simulink model "simulink_flightgear_control_trim_wind_5"  (R2023a)
settings: Solver=VariableStepAuto  StartTime=0  StopTime=inf  FixedStep=0.1  RelTol=1e-3
values from neighbouring files (symbols this model uses):
  alpha = -5:0.1:25    [Boeing747model.m]
  alpha1 = 0:0.1:14    [Boeing747model.m]
  alpha2 = -5:0.1:25    [Boeing747model.m]
  alpha3 = -5:0.1:17    [Boeing747model.m]
  beta = -15:0.1:15    [Boeing747model.m]
  CL = 0:0.01:1.4    [Boeing747model.m]
  da = 0:1:20    [Boeing747model.m]
  dr = [0 5 10 15 20 25]    [Boeing747model.m]
  EPR_ = 0:0.1:1.8    [Boeing747model.m]    (also in engine.m)
  flap = [0 10 20 25 30]    [Boeing747model.m]
  high1 = 0:10000:40000    [Boeing747model.m]
  high2 = 0:20000:40000    [Boeing747model.m]
  high3 = [0 15000 25000 35000 40000]    [Boeing747model.m]    (also in engine.m)
  high4 = [0 10000 20000 40000]    [Boeing747model.m]
  interp_result = table2array(resultTable(:,2:end))    [Boeing747model.m]
  interp_result_mach = 0:0.1:0.9    [Boeing747model.m]
  interp_result_N1 = 80:5:110    [Boeing747model.m]
  m2ft = 3.280839895013    (= 3.28083989501)    [Boeing747model.m]    (also in engine.m)
  mach = 0:0.02:0.9    [Boeing747model.m]    (also in engine.m)
  mach1 = [0 0.3 0.5 0.7 0.8 0.84 0.86 0.88 0.9]    [Boeing747model.m]
  mach2 = [0 0.3 0.5 0.7 0.8 0.9]    [Boeing747model.m]
  mach3 = [0 0.1 0.3 0.5 0.6 0.7 0.8 0.9]    [Boeing747model.m]    (also in engine.m = [0 0.1 0.3 0.5  0.7 0.8 0.9])
  mach5 = [0 0.6 0.8 0.85 0.9]    [Boeing747model.m]
  mach6 = [0 0.6 0.8 0.9]    [Boeing747model.m]
  mach7 = [0 0.3 0.5 0.74 0.8 0.84 0.86 0.88 0.9]    [Boeing747model.m]
  mach8 = [0 0.3 0.5 0.74 0.8 0.84 0.86 0.88 0.9]    [Boeing747model.m]
  model = 'simulink_flightgear_control_trim_wind_5'    [traimcode.m]
  ms2kts = 1.943844492609    (= 1.94384449261)    [Boeing747model.m]    (also in engine.m)
  powerangle_ = 0:1:130    [Boeing747model.m]    (also in engine.m)
  T = [-45 0 60 120]    [Boeing747model.m]    (also in engine.m)
  V_E = 0:20:250    [Boeing747model.m]
undefined symbols (not defined in the file or in its folder): Earth, F, ft, Light, m, MIL, Model, Newton, P3DAERO, Raphson, Receive, s, Send, Unit, WGS84, Wind
libraries: simulink_extras x115, aerolibconvert2 x16, simulink x4, aerolibfltsims x3, shared6dof x1, aerolibasang x1, aerolibtransform2 x1, aerolibatmos2 x1, aerolibobsolete x1, aerolibwind2 x1
(part 3 of 5)

== system simulink_flightgear_control_trim_wind_5/Plane/参数计算/航迹角/Subsystem3 ==
  Vg : Inport
  Demux2 : Demux  Outputs=3
  Product : Product  RndMeth=Zero
  Product1 : Product  RndMeth=Zero
  Sum : Sum  Inputs=++|
  Terminator1 : Terminator
  Vx²+Vy² : Outport  VectorParamsAs1DForOutWhenUnconnected=off
  wires:
  Product1/1 -> Sum/2
  Demux2/1 -> Product/1, Product/2
  Vg/1 -> Demux2/1
  Demux2/2 -> Product1/1, Product1/2
  Product/1 -> Sum/1
  Sum/1 -> Vx²+Vy²/1
  Demux2/3 -> Terminator1/1

== system simulink_flightgear_control_trim_wind_5/Plane/大气环境/风场_地面坐标系/Subsystem ==
  Vgx : Inport
  WindSpeed : Inport  Port=2
  Abs : Abs  SaturateOnIntegerOverflow=off
  Constant2 : Constant  Value=Wind.Total.Length
  Divide : Product  Inputs=*/
  Rate Limiter Dynamic : simulink/Discontinuities/Rate Limiter Dynamic
  Saturation : Saturate  UpperLimit=inf  LowerLimit=Wind.Total.GrowRate_Min
  Saturation1 : Saturate  UpperLimit=-Wind.Total.GrowRate_Min  LowerLimit=-inf
  Unary Minus : UnaryMinus
  V_Wind : Outport  VectorParamsAs1DForOutWhenUnconnected=off
  wires:
  Saturation1/1 -> Rate Limiter Dynamic/3
  Saturation/1 -> Rate Limiter Dynamic/1
  Abs/1 -> Divide/1
  Unary Minus/1 -> Saturation1/1
  Vgx/1 -> Abs/1
  Divide/1 -> Saturation/1, Unary Minus/1
  Constant2/1 -> Divide/2
  WindSpeed/1 -> Rate Limiter Dynamic/2
  Rate Limiter Dynamic/1 -> V_Wind/1

== system simulink_flightgear_control_trim_wind_5/Plane/大气环境/风场_地面坐标系/常值风 ==
  h(m) : Inport
  Constant : Constant  Value=0
  Fcn : Fcn  Expr=Wind.Constant.Vxy_Ground + (Wind.Constant.Vxy_RefAlt / Wind.Constant.RefAlt^2)
  Gain : Gain  Gain=cos(deg2rad(Wind.Constant.Direction))
  Gain1 : Gain  Gain=sin(deg2rad(Wind.Constant.Direction))
  Mux : Mux  Inputs=3
  V_Wind_Constant : Outport  VectorParamsAs1DForOutWhenUnconnected=off
  wires:
  Mux/1 -> V_Wind_Constant/1
  Gain1/1 -> Mux/2
  Constant/1 -> Mux/3
  Fcn/1 -> Gain/1, Gain1/1
  Gain/1 -> Mux/1
  h(m)/1 -> Fcn/1

== system simulink_flightgear_control_trim_wind_5/Plane/大气环境/风场_地面坐标系/自定义 ==
  Angle Conversion2 : aerolibconvert2/Angle Conversion  IU=deg  OU=rad
  Mux : Mux  Inputs=3
  Product : Product
  Product1 : Product
  Trigonometric Function : Trigonometry  Operator=cos
  Trigonometric Function1 : Trigonometry
  Wind_Custom_Direction : Constant  Value=Wind.Custom.Direction
  Wind_Custom_Vxy : Constant  Value=Wind.Custom.Vxy
  Wind_Custom_Vz : Constant  Value=Wind.Custom.Vz
  V_Wind_Custom : Outport  VectorParamsAs1DForOutWhenUnconnected=off
  wires:
  Angle Conversion2/1 -> Trigonometric Function/1, Trigonometric Function1/1
  Wind_Custom_Vxy/1 -> Product/1, Product1/1
  Trigonometric Function/1 -> Product/2
  Trigonometric Function1/1 -> Product1/2
  Wind_Custom_Direction/1 -> Angle Conversion2/1
  Product/1 -> Mux/1
  Wind_Custom_Vz/1 -> Mux/3
  Product1/1 -> Mux/2
  Mux/1 -> V_Wind_Custom/1

== system simulink_flightgear_control_trim_wind_5/Plane/大气环境/风场_地面坐标系/阵风 ==
  Angle Conversion1 : aerolibconvert2/Angle Conversion  IU=deg  OU=rad
  Constant1 : Constant  Value=Wind.Gust.Vxy_max
  Constant2 : Constant  Value=Wind.Gust.Vz_max
  Constant3 : Constant  Value=Wind.Gust.Act_Random_V
  Constant4 : Constant  Value=Wind.Gust.Direction
  Constant6 : Constant  Value=Wind.Gust.Act_Random_Direction
  Constant7 : Constant  Value=Wind.Gust.Act_Random_V
  Mux : Mux  Inputs=3
  Product : Product
  Product3 : Product
  Product4 : Product
  Pulse Generator : DiscretePulseGenerator  PulseType=Time based  Period=Wind.Gust.SampleTime + Wind.Gust.ContinueTime  PulseWidth=Wind.Gust.ContinueTime / (Wind.Gust.SampleTime + Wind.Gust.ContinueTime) * 100  PhaseDelay=Wind.Gust.SampleTime
  Switch : Switch  Criteria=u2 ~= 0  SaturateOnIntegerOverflow=off  InputSameDT=off
  Switch1 : Switch  Criteria=u2 ~= 0  SaturateOnIntegerOverflow=off  InputSameDT=off
  Switch2 : Switch  Criteria=u2 ~= 0  SaturateOnIntegerOverflow=off  InputSameDT=off
  Trigonometric Function : Trigonometry  Operator=cos
  Trigonometric Function1 : Trigonometry
  Uniform Random Number : UniformRandomNumber  Minimum=Wind.Gust.Vxy_min  Maximum=Wind.Gust.Vxy_max + eps  Seed=fix(rand(1,1)*25000)  SampleTime=Wind.Gust.SampleTime + Wind.Gust.ContinueTime
  Uniform Random Number1 : UniformRandomNumber  Minimum=0  Maximum=360  Seed=fix(rand(1,1)*25000)  SampleTime=Wind.Gust.SampleTime + Wind.Gust.ContinueTime
  Uniform Random Number2 : UniformRandomNumber  Minimum=Wind.Gust.Vz_min  Maximum=Wind.Gust.Vz_max + eps  Seed=fix(rand(1,1)*25000)  SampleTime=Wind.Gust.SampleTime + Wind.Gust.ContinueTime
  V_Wind_Gust : Outport  VectorParamsAs1DForOutWhenUnconnected=off
  wires:
  Uniform Random Number2/1 -> Switch2/1
  Constant7/1 -> Switch2/2
  Angle Conversion1/1 -> Trigonometric Function/1, Trigonometric Function1/1
  Constant4/1 -> Switch1/3
  Uniform Random Number1/1 -> Switch1/1
  Constant6/1 -> Switch1/2
  Trigonometric Function1/1 -> Product4/2
  Trigonometric Function/1 -> Product/2
  Switch/1 -> Product/1, Product4/1
  Switch1/1 -> Angle Conversion1/1
  Mux/1 -> Product3/1
  Constant2/1 -> Switch2/3
  Constant3/1 -> Switch/2
  Switch2/1 -> Mux/3
  Uniform Random Number/1 -> Switch/1
  Constant1/1 -> Switch/3
  Pulse Generator/1 -> Product3/2
  Product4/1 -> Mux/2
  Product/1 -> Mux/1
  Product3/1 -> V_Wind_Gust/1

== system simulink_flightgear_control_trim_wind_5/Plane/气动系数/Subsystem58/Subsystem ==
  note: 高速模式
  In1 : Inport
  Radians in : Inport  Port=2
  In3 : Inport  Port=3
  2-D Lookup Table3 : Lookup_n-D  BreakpointsForDimension1=mach7  BreakpointsForDimension2=alpha2  Table=P3DAERO.CL_mach  InternalRulePriority=Speed  RndMeth=Simplest
      settings: InputPortMap=u0,u1
  Radians to Degrees : simulink_extras/Transformations/Radians to Degrees
  Scope2 : Scope
  Out1 : Outport
  wires:
  Radians in/1 -> Radians to Degrees/1
  Radians to Degrees/1 -> 2-D Lookup Table3/2
  In3/1 -> 2-D Lookup Table3/1
  2-D Lookup Table3/1 -> Scope2/1, Out1/1

== system simulink_flightgear_control_trim_wind_5/Plane/气动系数/Subsystem58/Subsystem1 ==
  note: 高速模式
  note: 低速模式
  In1 : Inport
  In2 : Inport  Port=2
  In3 : Inport  Port=3
  In4 : Inport  Port=4
  2-D Lookup Table19 : Lookup_n-D  BreakpointsForDimension1=flap  BreakpointsForDimension2=V_E  Table=P3DAERO.Delta_CL_lowspeed  InternalRulePriority=Speed  RndMeth=Simplest
      settings: InputPortMap=u0,u1
  2-D Lookup Table20 : Lookup_n-D  BreakpointsForDimension1=high1  BreakpointsForDimension2=mach  Table=P3DAERO.Delta_CL_highspeed  InternalRulePriority=Speed  RndMeth=Simplest
      settings: InputPortMap=u0,u1
  Gain11 : Gain  Gain=-1
  Scope6 : Scope
  Velocity Conversion : aerolibconvert2/Velocity Conversion  IU=m/s  OU=ft/s
  Out1 : Outport
  wires:
  2-D Lookup Table20/1 -> Gain11/1
  Gain11/1 -> Out1/1, Scope6/1
  In4/1 -> 2-D Lookup Table20/2
  In2/1 -> 2-D Lookup Table19/2
  In3/1 -> Velocity Conversion/1
  In1/1 -> 2-D Lookup Table19/1
  Velocity Conversion/1 -> 2-D Lookup Table20/1

== system simulink_flightgear_control_trim_wind_5/Plane/气动系数/Subsystem58/Subsystem10 ==
  note: dot_CL_dot_delta_ei
  In1 : Inport
  In2 : Inport  Port=2
  In3 : Inport  Port=3
  Radians in : Inport  Port=4
  2-D Lookup Table10 : Lookup_n-D  BreakpointsForDimension1=high1  BreakpointsForDimension2=mach  Table=P3DAERO.dot_CL_dot_delta_ei  InternalRulePriority=Speed  RndMeth=Simplest
      settings: InputPortMap=u0,u1
  Gain : Gain
  Product6 : Product  Inputs=3
  Radians to Degrees4 : simulink_extras/Transformations/Radians to Degrees
  Scope1 : Scope
  Scope18 : Scope
  Velocity Conversion : aerolibconvert2/Velocity Conversion  IU=m/s  OU=ft/s
  Out1 : Outport
  wires:
  Product6/1 -> Gain/1, Scope18/1
  Radians in/1 -> Radians to Degrees4/1
  In1/1 -> Product6/1
  Radians to Degrees4/1 -> Product6/3, Scope1/1
  2-D Lookup Table10/1 -> Product6/2
  In3/1 -> 2-D Lookup Table10/2
  In2/1 -> Velocity Conversion/1
  Gain/1 -> Out1/1
  Velocity Conversion/1 -> 2-D Lookup Table10/1

== system simulink_flightgear_control_trim_wind_5/Plane/气动系数/Subsystem58/Subsystem12 ==
  In1 : Inport
  Radians in : Inport  Port=2
  2-D Lookup Table : Lookup_n-D  BreakpointsForDimension1=flap  BreakpointsForDimension2=alpha  Table=P3DAERO.CD_basic  InternalRulePriority=Speed  RndMeth=Simplest
      settings: InputPortMap=u0,u1
  Radians to Degrees : simulink_extras/Transformations/Radians to Degrees
  Scope14 : Scope
  Out1 : Outport
  wires:
  In1/1 -> 2-D Lookup Table/1
  Radians to Degrees/1 -> 2-D Lookup Table/2
  2-D Lookup Table/1 -> Out1/1, Scope14/1
  Radians in/1 -> Radians to Degrees/1

== system simulink_flightgear_control_trim_wind_5/Plane/气动系数/Subsystem58/Subsystem13 ==
  In1 : Inport
  Radians in : Inport  Port=2
  Radians in1 : Inport  Port=3
  2-D Lookup Table1 : Lookup_n-D  BreakpointsForDimension1=flap  BreakpointsForDimension2=alpha  Table=P3DAERO.dot_CD_dot_delta  InternalRulePriority=Speed  RndMeth=Simplest
      settings: InputPortMap=u0,u1
  Product : Product
  Radians to Degrees2 : simulink_extras/Transformations/Radians to Degrees
  Radians to Degrees7 : simulink_extras/Transformations/Radians to Degrees
  Scope5 : Scope
  Out1 : Outport
  wires:
  Radians in1/1 -> Radians to Degrees2/1
  Product/1 -> Out1/1, Scope5/1
  Radians to Degrees2/1 -> Product/2
  2-D Lookup Table1/1 -> Product/1
  Radians to Degrees7/1 -> 2-D Lookup Table1/2
  In1/1 -> 2-D Lookup Table1/1
  Radians in/1 -> Radians to Degrees7/1

== system simulink_flightgear_control_trim_wind_5/Plane/气动系数/Subsystem58/Subsystem14 ==
  In1 : Inport
  In2 : Inport  Port=2
  In3 : Inport  Port=3
  In4 : Inport  Port=4
  In5 : Inport  Port=5
  2-D Lookup Table2 : Lookup_n-D  BreakpointsForDimension1=mach1  BreakpointsForDimension2=CL  Table=P3DAERO.CD_mach  InternalRulePriority=Speed  RndMeth=Simplest
      settings: InputPortMap=u0,u1
  Gain : Gain
  Scope : Scope
  Scope2 : Scope
  Sum2 : Sum
  Out1 : Outport
  wires:
  In4/1 -> 2-D Lookup Table2/1
  2-D Lookup Table2/1 -> Gain/1
  In5/1 -> 2-D Lookup Table2/2
  Gain/1 -> Scope/1, Out1/1
  Sum2/1 -> Scope2/1
  In1/1 -> Sum2/1
  In2/1 -> Sum2/2

== system simulink_flightgear_control_trim_wind_5/Plane/气动系数/Subsystem58/Subsystem15 ==
  Radians in : Inport
  In2 : Inport  Port=2
  2-D Lookup Table6 : Lookup_n-D  BreakpointsForDimension1=dr  BreakpointsForDimension2=beta  Table=P3DAERO.delta_CD_25R  InternalRulePriority=Speed  RndMeth=Simplest
      settings: InputPortMap=u0,u1
  2-D Lookup Table9 : Lookup_n-D  BreakpointsForDimension1=dr  BreakpointsForDimension2=beta  Table=P3DAERO.delta_CD_fu25R  InternalRulePriority=Speed  RndMeth=Simplest
      settings: InputPortMap=u0,u1
  Abs1 : Abs  SaturateOnIntegerOverflow=off
  Gain4 : Gain  Gain=0.6
  Gain8 : Gain  Gain=0.6
  Radians to Degrees{6,8..9,11} (4 alike) : simulink_extras/Transformations/Radians to Degrees
  Saturation1 : Saturate  UpperLimit=15  LowerLimit=-15
  Saturation9 : Saturate  UpperLimit=15  LowerLimit=-15
  Scope17 : Scope
  Switch2 : Switch  SaturateOnIntegerOverflow=off  InputSameDT=off
  Out1 : Outport
  wires:
  Radians to Degrees9/1 -> Abs1/1
  Radians in/1 -> Radians to Degrees8/1, Radians to Degrees6/1
  In2/1 -> Radians to Degrees9/1, Radians to Degrees11/1, Switch2/2
  2-D Lookup Table6/1 -> Gain4/1, Scope17/1
  Gain4/1 -> Switch2/1
  Gain8/1 -> Switch2/3
  Saturation9/1 -> 2-D Lookup Table6/2
  Radians to Degrees6/1 -> Saturation9/1
  2-D Lookup Table9/1 -> Gain8/1
  Radians to Degrees8/1 -> Saturation1/1
  Radians to Degrees11/1 -> 2-D Lookup Table6/1
  Switch2/1 -> Out1/1
  Abs1/1 -> 2-D Lookup Table9/1
  Saturation1/1 -> 2-D Lookup Table9/2

== system simulink_flightgear_control_trim_wind_5/Plane/气动系数/Subsystem58/Subsystem16 ==
  Radians in : Inport
  In2 : Inport  Port=2
  2-D Lookup Table7 : Lookup_n-D  BreakpointsForDimension1=dr  BreakpointsForDimension2=beta  Table=P3DAERO.delta_CD_25R  InternalRulePriority=Speed  RndMeth=Simplest
      settings: InputPortMap=u0,u1
  2-D Lookup Table8 : Lookup_n-D  BreakpointsForDimension1=dr  BreakpointsForDimension2=beta  Table=P3DAERO.delta_CD_fu25R  InternalRulePriority=Speed  RndMeth=Simplest
      settings: InputPortMap=u0,u1
  Abs2 : Abs  SaturateOnIntegerOverflow=off
  Gain10 : Gain  Gain=0.4
  Gain12 : Gain  Gain=0.4
  Radians to Degrees{5,10,12..13} (4 alike) : simulink_extras/Transformations/Radians to Degrees
  Saturation1 : Saturate  UpperLimit=15  LowerLimit=-15
  Saturation10 : Saturate  UpperLimit=15  LowerLimit=-15
  Scope11 : Scope
  Switch3 : Switch  SaturateOnIntegerOverflow=off  InputSameDT=off
  Out1 : Outport
  wires:
  Gain10/1 -> Scope11/1, Switch3/1
  Radians in/1 -> Radians to Degrees12/1, Radians to Degrees5/1
  Radians to Degrees12/1 -> Saturation1/1
  In2/1 -> Radians to Degrees13/1, Radians to Degrees10/1, Switch3/2
  Radians to Degrees13/1 -> Abs2/1
  Gain12/1 -> Switch3/3
  Saturation10/1 -> 2-D Lookup Table7/2
  2-D Lookup Table7/1 -> Gain10/1
  Radians to Degrees5/1 -> Saturation10/1
  Radians to Degrees10/1 -> 2-D Lookup Table7/1
  2-D Lookup Table8/1 -> Gain12/1
  Switch3/1 -> Out1/1
  Abs2/1 -> 2-D Lookup Table8/1
  Saturation1/1 -> 2-D Lookup Table8/2

== system simulink_flightgear_control_trim_wind_5/Plane/气动系数/Subsystem58/Subsystem17 ==
  note: 米变英尺
  In1 : Inport
  In2 : Inport  Port=2
  Radians in : Inport  Port=3
  1-D Lookup Table97 : Lookup_n-D  NumberOfTableDimensions=1  BreakpointsForDimension1=P3DAERO.k_ge_A(1,:)  Table=P3DAERO.k_ge_A(2,:)  InternalRulePriority=Speed  RndMeth=Simplest
  2-D Lookup Table4 : Lookup_n-D  BreakpointsForDimension1=flap  BreakpointsForDimension2=alpha1  Table=P3DAERO.delta_CD_ge  InternalRulePriority=Speed  RndMeth=Simplest
      settings: InputPortMap=u0,u1
  Constant24 : Constant  Value=0
  Gain : Gain
  Product1 : Product
  Radians to Degrees3 : simulink_extras/Transformations/Radians to Degrees
  Saturation1 : Saturate  UpperLimit=14  LowerLimit=0
  Scope15 : Scope
  Scope49 : Scope
  Switch12 : Switch  Criteria=u2 > Threshold  Threshold=24  SaturateOnIntegerOverflow=off  InputSameDT=off
  Velocity Conversion : aerolibconvert2/Velocity Conversion  IU=m/s  OU=ft/s
  Out1 : Outport
  wires:
  Saturation1/1 -> 2-D Lookup Table4/2
  Switch12/1 -> Gain/1, Scope49/1
  Radians to Degrees3/1 -> Saturation1/1
  1-D Lookup Table97/1 -> Product1/1
  Velocity Conversion/1 -> 1-D Lookup Table97/1
  Product1/1 -> Switch12/3
  Radians in/1 -> Radians to Degrees3/1
  2-D Lookup Table4/1 -> Scope15/1, Product1/2
  In2/1 -> 2-D Lookup Table4/1
  Constant24/1 -> Switch12/1
  Gain/1 -> Out1/1
  In1/1 -> Switch12/2, Velocity Conversion/1

== system simulink_flightgear_control_trim_wind_5/Plane/气动系数/Subsystem58/Subsystem18 ==
  In1 : Inport
  Radians in : Inport  Port=2
  2-D Lookup Table5 : Lookup_n-D  BreakpointsForDimension1=flap  BreakpointsForDimension2=beta  Table=P3DAERO.delta_CD_sideslip  InternalRulePriority=Speed  RndMeth=Simplest
      settings: InputPortMap=u0,u1
  Gain1 : Gain  Gain=-1
  Radians to Degrees4 : simulink_extras/Transformations/Radians to Degrees
  Saturation8 : Saturate  UpperLimit=15  LowerLimit=-15
  Scope16 : Scope
  Out1 : Outport
  wires:
  Gain1/1 -> Out1/1, Scope16/1
  Radians to Degrees4/1 -> Saturation8/1
  Saturation8/1 -> 2-D Lookup Table5/2
  In1/1 -> 2-D Lookup Table5/1
  2-D Lookup Table5/1 -> Gain1/1
  Radians in/1 -> Radians to Degrees4/1

== system simulink_flightgear_control_trim_wind_5/Plane/气动系数/Subsystem58/Subsystem19 ==
  In1 : Inport
  In2 : Inport  Port=2
  Radians in : Inport  Port=3
  In4 : Inport  Port=4
  1-D Lookup Table91 : Lookup_n-D  NumberOfTableDimensions=1  BreakpointsForDimension1=P3DAERO.CD_mach_gear(1,:)  Table=P3DAERO.CD_mach_gear(2,:)  InternalRulePriority=Speed  RndMeth=Simplest
  2-D Lookup Table3 : Lookup_n-D  BreakpointsForDimension1=flap  BreakpointsForDimension2=alpha  Table=P3DAERO.delta_CD_gear  InternalRulePriority=Speed  RndMeth=Simplest
      settings: InputPortMap=u0,u1
  Product15 : Product  Inputs=3
  Radians to Degrees2 : simulink_extras/Transformations/Radians to Degrees
  Scope17 : Scope
  Scope47 : Scope
  Out1 : Outport
  wires:
  Product15/1 -> Out1/1, Scope47/1
  In2/1 -> 2-D Lookup Table3/1
  2-D Lookup Table3/1 -> Product15/2
  Radians to Degrees2/1 -> 2-D Lookup Table3/2
  In1/1 -> Product15/1
  1-D Lookup Table91/1 -> Scope17/1, Product15/3
  In4/1 -> 1-D Lookup Table91/1
  Radians in/1 -> Radians to Degrees2/1

== system simulink_flightgear_control_trim_wind_5/Plane/气动系数/Subsystem58/Subsystem2 ==
  note: dot_CL_dot_delta_eo
  In1 : Inport
  In2 : Inport  Port=2
  In3 : Inport  Port=3
  Radians in : Inport  Port=4
  2-D Lookup Table11 : Lookup_n-D  BreakpointsForDimension1=high1  BreakpointsForDimension2=mach  Table=P3DAERO.dot_CL_dot_delta_eo  InternalRulePriority=Speed  RndMeth=Simplest
      settings: InputPortMap=u0,u1
  Gain : Gain
  Product7 : Product  Inputs=3
  Radians to Degrees5 : simulink_extras/Transformations/Radians to Degrees
  Scope1 : Scope
  Scope19 : Scope
  Velocity Conversion : aerolibconvert2/Velocity Conversion  IU=m/s  OU=ft/s
  Out1 : Outport
  wires:
  Radians to Degrees5/1 -> Scope1/1, Product7/3
  In3/1 -> 2-D Lookup Table11/2
  Product7/1 -> Gain/1, Scope19/1
  In1/1 -> Product7/1
  2-D Lookup Table11/1 -> Product7/2
  Radians in/1 -> Radians to Degrees5/1
  In2/1 -> Velocity Conversion/1
  Gain/1 -> Out1/1
  Velocity Conversion/1 -> 2-D Lookup Table11/1

== system simulink_flightgear_control_trim_wind_5/Plane/气动系数/Subsystem58/Subsystem20 ==
  In1 : Inport
  Radians in : Inport  Port=2
  In3 : Inport  Port=3
  2-D Lookup Table : Lookup_n-D  BreakpointsForDimension1=flap  BreakpointsForDimension2=alpha  Table=P3DAERO.Cm_25_basic  InternalRulePriority=Speed  RndMeth=Simplest
      settings: InputPortMap=u0,u1
  2-D Lookup Table1 : Lookup_n-D  BreakpointsForDimension1=mach8  BreakpointsForDimension2=alpha3  Table=P3DAERO.Cm_mach  InternalRulePriority=Speed  RndMeth=Simplest
      settings: InputPortMap=u0,u1
  Radians to Degrees6 : simulink_extras/Transformations/Radians to Degrees
  Saturation : Saturate  UpperLimit=17  LowerLimit=-5
  Scope : Scope
  Scope2 : Scope
  Scope3 : Scope
  Out1 : Outport
  wires:
  Saturation/1 -> Scope3/1, 2-D Lookup Table1/2
  In3/1 -> 2-D Lookup Table1/1
  In1/1 -> 2-D Lookup Table/1
  2-D Lookup Table1/1 -> Scope2/1, Out1/1
  Radians in/1 -> Radians to Degrees6/1
  Radians to Degrees6/1 -> Saturation/1, 2-D Lookup Table/2
  2-D Lookup Table/1 -> Scope/1

== system simulink_flightgear_control_trim_wind_5/Plane/气动系数/Subsystem58/Subsystem21 ==
  note: 低速模式
  note: 高速模式
  In1 : Inport
  In2 : Inport  Port=2
  In3 : Inport  Port=3
  In4 : Inport  Port=4
  2-D Lookup Table1 : Lookup_n-D  BreakpointsForDimension1=high1  BreakpointsForDimension2=mach  Table=P3DAERO.delta_Cm_25_highspeed  InternalRulePriority=Speed  RndMeth=Simplest
      settings: InputPortMap=u0,u1
  2-D Lookup Table2 : Lookup_n-D  BreakpointsForDimension1=flap  BreakpointsForDimension2=V_E  Table=P3DAERO.delta_Cm_25_lowspeed  InternalRulePriority=Speed  RndMeth=Simplest
      settings: InputPortMap=u0,u1
  Gain7 : Gain  Gain=m2ft
  Scope2 : Scope
  Out1 : Outport
  wires:
  In2/1 -> 2-D Lookup Table2/2
  Gain7/1 -> 2-D Lookup Table1/1
  In3/1 -> Gain7/1
  In1/1 -> 2-D Lookup Table2/1
  2-D Lookup Table1/1 -> Out1/1, Scope2/1
  In4/1 -> 2-D Lookup Table1/2

== system simulink_flightgear_control_trim_wind_5/Plane/气动系数/Subsystem58/Subsystem22 ==
  note: 地效修正
  note: 米变英尺
  In1 : Inport
  In2 : Inport  Port=2
  Radians in : Inport  Port=3
  1-D Lookup Table97 : Lookup_n-D  NumberOfTableDimensions=1  BreakpointsForDimension1=P3DAERO.k_ge(1,:)  Table=P3DAERO.k_ge(2,:)  InternalRulePriority=Speed  RndMeth=Simplest
  2-D Lookup Table13 : Lookup_n-D  BreakpointsForDimension1=flap  BreakpointsForDimension2=alpha1  Table=P3DAERO.Fm  InternalRulePriority=Speed  RndMeth=Simplest
      settings: InputPortMap=u0,u1
  Constant21 : Constant
  Gain14 : Gain  Gain=m2ft
  Product16 : Product
  Radians to Degrees2 : simulink_extras/Transformations/Radians to Degrees
  Saturation : Saturate  UpperLimit=14  LowerLimit=0
  Scope31 : Scope
  Scope48 : Scope
  Sum11 : Sum
  Switch5 : Switch  Criteria=u2 > Threshold  Threshold=24  SaturateOnIntegerOverflow=off  InputSameDT=off
  Out1 : Outport
  wires:
  Saturation/1 -> 2-D Lookup Table13/2
  Gain14/1 -> 1-D Lookup Table97/1
  Product16/1 -> Sum11/2
  Switch5/1 -> Out1/1, Scope31/1
  Radians to Degrees2/1 -> Saturation/1
  2-D Lookup Table13/1 -> Product16/2
  Sum11/1 -> Switch5/3
  Radians in/1 -> Radians to Degrees2/1
  Constant21/1 -> Sum11/1, Switch5/1
  1-D Lookup Table97/1 -> Scope48/1, Product16/1
  In2/1 -> 2-D Lookup Table13/1
  In1/1 -> Switch5/2, Gain14/1

== system simulink_flightgear_control_trim_wind_5/Plane/气动系数/Subsystem58/Subsystem23 ==
  In1 : Inport
  Radians in : Inport  Port=2
  In3 : Inport  Port=3
  Radians in1 : Inport  Port=4
  In5 : Inport  Port=5
  1-D Lookup Table1 : Lookup_n-D  NumberOfTableDimensions=1  BreakpointsForDimension1=P3DAERO.delta_CM_25_ai_flapup(1,:)  Table=P3DAERO.delta_CM_25_ai_flapup(2,:)  InternalRulePriority=Speed  RndMeth=Simplest
  1-D Lookup Table2 : Lookup_n-D  NumberOfTableDimensions=1  BreakpointsForDimension1=P3DAERO.delta_CM_25_ai_flapdown(1,:)  Table=P3DAERO.delta_CM_25_ai_flapdown(2,:)  InternalRulePriority=Speed  RndMeth=Simplest
  1-D Lookup Table35 : Lookup_n-D  NumberOfTableDimensions=1  BreakpointsForDimension1=P3DAERO.delta_CM_25_ai_mach(1,:)  Table=P3DAERO.delta_CM_25_ai_mach(2,:)  InternalRulePriority=Speed  RndMeth=Simplest
  2-D Lookup Table14 : Lookup_n-D  BreakpointsForDimension1=flap  BreakpointsForDimension2=da  Table=P3DAERO.k_delta_ai  InternalRulePriority=Speed  RndMeth=Simplest
      settings: InputPortMap=u0,u1
  Product4 : Product  Inputs=4
  Radians to Degrees4 : simulink_extras/Transformations/Radians to Degrees
  Radians to Degrees8 : simulink_extras/Transformations/Radians to Degrees
  Saturation2 : Saturate  UpperLimit=20  LowerLimit=0
  Scope15 : Scope
  Switch15 : Switch  Criteria=u2 ~= 0  Threshold=0.35  SaturateOnIntegerOverflow=off  InputSameDT=off
  Out1 : Outport
  wires:
  Radians to Degrees4/1 -> Saturation2/1
  1-D Lookup Table1/1 -> Switch15/3
  1-D Lookup Table2/1 -> Switch15/1
  2-D Lookup Table14/1 -> Product4/3
  Switch15/1 -> Product4/2
  In1/1 -> 1-D Lookup Table35/1
  Saturation2/1 -> 2-D Lookup Table14/2
  In3/1 -> Switch15/2, 2-D Lookup Table14/1
  Product4/1 -> Out1/1, Scope15/1
  Radians to Degrees8/1 -> 1-D Lookup Table2/1, 1-D Lookup Table1/1
  In5/1 -> Product4/4
  1-D Lookup Table35/1 -> Product4/1
  Radians in/1 -> Radians to Degrees8/1
  Radians in1/1 -> Radians to Degrees4/1

== system simulink_flightgear_control_trim_wind_5/Plane/气动系数/Subsystem58/Subsystem24 ==
  In1 : Inport
  Radians in : Inport  Port=2
  In3 : Inport  Port=3
  Radians in1 : Inport  Port=4
  In5 : Inport  Port=5
  1-D Lookup Table3 : Lookup_n-D  NumberOfTableDimensions=1  BreakpointsForDimension1=P3DAERO.delta_CM_25_ai_flapup(1,:)  Table=P3DAERO.delta_CM_25_ai_flapup(2,:)  InternalRulePriority=Speed  RndMeth=Simplest
  1-D Lookup Table4 : Lookup_n-D  NumberOfTableDimensions=1  BreakpointsForDimension1=P3DAERO.delta_CM_25_ai_flapdown(1,:)  Table=P3DAERO.delta_CM_25_ai_flapdown(2,:)  InternalRulePriority=Speed  RndMeth=Simplest
  1-D Lookup Table5 : Lookup_n-D  NumberOfTableDimensions=1  BreakpointsForDimension1=P3DAERO.delta_CM_25_ai_mach(1,:)  Table=P3DAERO.delta_CM_25_ai_mach(2,:)  InternalRulePriority=Speed  RndMeth=Simplest
  2-D Lookup Table15 : Lookup_n-D  BreakpointsForDimension1=flap  BreakpointsForDimension2=da  Table=P3DAERO.k_delta_ai  InternalRulePriority=Speed  RndMeth=Simplest
      settings: InputPortMap=u0,u1
  Product18 : Product  Inputs=4
  Radians to Degrees16 : simulink_extras/Transformations/Radians to Degrees
  Radians to Degrees9 : simulink_extras/Transformations/Radians to Degrees
  Saturation4 : Saturate  UpperLimit=20  LowerLimit=0
  Scope6 : Scope
  Switch16 : Switch  Criteria=u2 ~= 0  Threshold=0.35  SaturateOnIntegerOverflow=off  InputSameDT=off
  Out1 : Outport
  wires:
  Switch16/1 -> Product18/2
  Radians to Degrees9/1 -> Saturation4/1
  Saturation4/1 -> 2-D Lookup Table15/2
  1-D Lookup Table5/1 -> Product18/1
  In5/1 -> Product18/4
  1-D Lookup Table4/1 -> Switch16/1
  In3/1 -> 2-D Lookup Table15/1, Switch16/2
  Radians to Degrees16/1 -> 1-D Lookup Table4/1, 1-D Lookup Table3/1
  Product18/1 -> Out1/1, Scope6/1
  Radians in/1 -> Radians to Degrees16/1
  1-D Lookup Table3/1 -> Switch16/3
  2-D Lookup Table15/1 -> Product18/3
  In1/1 -> 1-D Lookup Table5/1
  Radians in1/1 -> Radians to Degrees9/1

== system simulink_flightgear_control_trim_wind_5/Plane/气动系数/Subsystem58/Subsystem25 ==
  note: 米变英尺
  In1 : Inport
  In2 : Inport  Port=2
  Radians in : Inport  Port=3
  1-D Lookup Table59 : Lookup_n-D  NumberOfTableDimensions=1  BreakpointsForDimension1=P3DAERO.k_ge(1,:)  Table=P3DAERO.k_ge(2,:)  InternalRulePriority=Speed  RndMeth=Simplest
  2-D Lookup Table21 : Lookup_n-D  BreakpointsForDimension1=flap  BreakpointsForDimension2=alpha1  Table=P3DAERO.delta_CM_25_ge  InternalRulePriority=Speed  RndMeth=Simplest
      settings: InputPortMap=u0,u1
  Constant24 : Constant  Value=0
  Gain3 : Gain  Gain=m2ft
  Product8 : Product
  Radians to Degrees14 : simulink_extras/Transformations/Radians to Degrees
  Saturation5 : Saturate  UpperLimit=14  LowerLimit=0
  Scope11 : Scope
  Scope49 : Scope
  Switch12 : Switch  Criteria=u2 > Threshold  Threshold=24  SaturateOnIntegerOverflow=off  InputSameDT=off
  Out1 : Outport
  wires:
  2-D Lookup Table21/1 -> Product8/2
  Constant24/1 -> Switch12/1
  Switch12/1 -> Out1/1, Scope49/1
  Radians to Degrees14/1 -> Saturation5/1
  Gain3/1 -> 1-D Lookup Table59/1
  1-D Lookup Table59/1 -> Product8/1, Scope11/1
  Product8/1 -> Switch12/3
  Saturation5/1 -> 2-D Lookup Table21/2
  Radians in/1 -> Radians to Degrees14/1
  In2/1 -> 2-D Lookup Table21/1
  In1/1 -> Switch12/2, Gain3/1

== system simulink_flightgear_control_trim_wind_5/Plane/气动系数/Subsystem58/Subsystem26 ==
  In1 : Inport
  Radians in : Inport  Port=2
  2-D Lookup Table22 : Lookup_n-D  BreakpointsForDimension1=flap  BreakpointsForDimension2=beta  Table=P3DAERO.delta_CM_25_sideslip  InternalRulePriority=Speed  RndMeth=Simplest
      settings: InputPortMap=u0,u1
  Radians to Degrees18 : simulink_extras/Transformations/Radians to Degrees
  Scope13 : Scope
  Out1 : Outport
  wires:
  In1/1 -> 2-D Lookup Table22/1
  2-D Lookup Table22/1 -> Out1/1, Scope13/1
  Radians to Degrees18/1 -> 2-D Lookup Table22/2
  Radians in/1 -> Radians to Degrees18/1

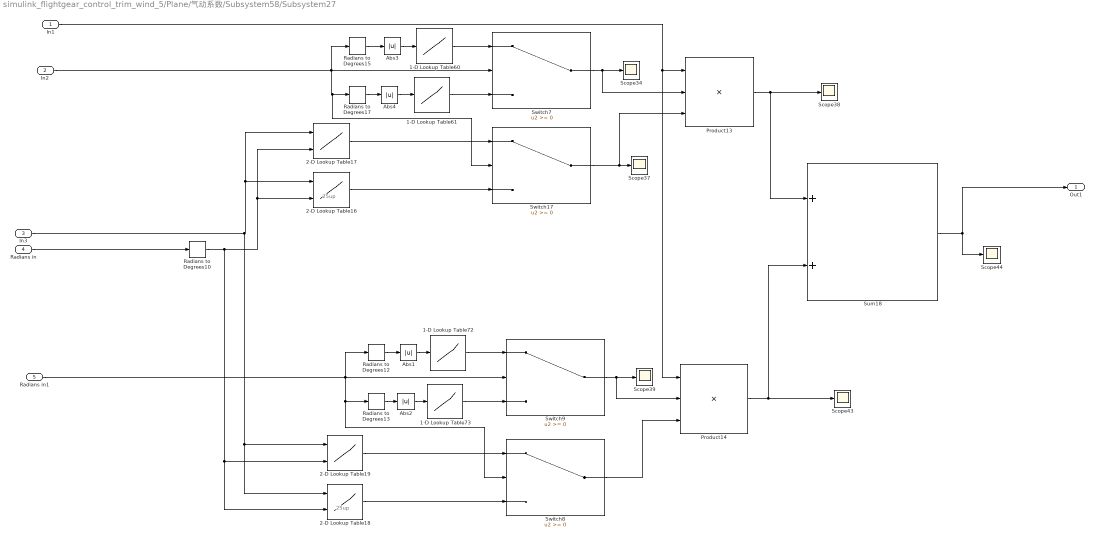
== system simulink_flightgear_control_trim_wind_5/Plane/气动系数/Subsystem58/Subsystem27 ==
  note: 25up
  note: 25up
  In1 : Inport
  In2 : Inport  Port=2
  In3 : Inport  Port=3
  Radians in : Inport  Port=4
  Radians in1 : Inport  Port=5
  1-D Lookup Table60 : Lookup_n-D  NumberOfTableDimensions=1  BreakpointsForDimension1=P3DAERO.k_delata_Ao_down(1,:)  Table=P3DAERO.k_delata_Ao_down(2,:)  InternalRulePriority=Speed  RndMeth=Simplest
  1-D Lookup Table61 : Lookup_n-D  NumberOfTableDimensions=1  BreakpointsForDimension1=P3DAERO.k_delata_Ao_up(1,:)  Table=P3DAERO.k_delata_Ao_up(2,:)  InternalRulePriority=Speed  RndMeth=Simplest
  1-D Lookup Table72 : Lookup_n-D  NumberOfTableDimensions=1  BreakpointsForDimension1=P3DAERO.k_delata_Ao_down(1,:)  Table=P3DAERO.k_delata_Ao_down(2,:)  InternalRulePriority=Speed  RndMeth=Simplest
  1-D Lookup Table73 : Lookup_n-D  NumberOfTableDimensions=1  BreakpointsForDimension1=P3DAERO.k_delata_Ao_up(1,:)  Table=P3DAERO.k_delata_Ao_up(2,:)  InternalRulePriority=Speed  RndMeth=Simplest
  2-D Lookup Table16 : Lookup_n-D  BreakpointsForDimension1=flap  BreakpointsForDimension2=alpha  Table=P3DAERO.delata_CM_25_Ao_25up  InternalRulePriority=Speed  RndMeth=Simplest
      settings: InputPortMap=u0,u1
  2-D Lookup Table17 : Lookup_n-D  BreakpointsForDimension1=flap  BreakpointsForDimension2=alpha  Table=P3DAERO.delata_CM_25_Ao_15down  InternalRulePriority=Speed  RndMeth=Simplest
      settings: InputPortMap=u0,u1
  2-D Lookup Table18 : Lookup_n-D  BreakpointsForDimension1=flap  BreakpointsForDimension2=alpha  Table=P3DAERO.delata_CM_25_Ao_25up  InternalRulePriority=Speed  RndMeth=Simplest
      settings: InputPortMap=u0,u1
  2-D Lookup Table19 : Lookup_n-D  BreakpointsForDimension1=flap  BreakpointsForDimension2=alpha  Table=P3DAERO.delata_CM_25_Ao_15down  InternalRulePriority=Speed  RndMeth=Simplest
      settings: InputPortMap=u0,u1
  Abs{1..4} (4 alike) : Abs  SaturateOnIntegerOverflow=off
  Product13 : Product  Inputs=3
  Product14 : Product  Inputs=3
  Radians to Degrees{10,12..13,15,17} (5 alike) : simulink_extras/Transformations/Radians to Degrees
  Scope{34,37..39,43..44} (6 alike) : Scope
  Sum18 : Sum
  Switch{7..9,17} (4 alike) : Switch  SaturateOnIntegerOverflow=off  InputSameDT=off
  Out1 : Outport
  wires:
  Abs2/1 -> 1-D Lookup Table73/1
  Abs3/1 -> 1-D Lookup Table60/1
  2-D Lookup Table16/1 -> Switch17/3
  Switch17/1 -> Scope37/1, Product13/3
  Radians in/1 -> Radians to Degrees10/1
  1-D Lookup Table60/1 -> Switch7/1
  Radians to Degrees15/1 -> Abs3/1
  Switch9/1 -> Product14/2, Scope39/1
  In1/1 -> Product13/1, Product14/1
  Product14/1 -> Scope43/1, Sum18/2
  Sum18/1 -> Out1/1, Scope44/1
  Radians to Degrees10/1 -> 2-D Lookup Table18/2, 2-D Lookup Table19/2, 2-D Lookup Table17/2, 2-D Lookup Table16/2
  1-D Lookup Table61/1 -> Switch7/3
  In3/1 -> 2-D Lookup Table19/1, 2-D Lookup Table18/1, 2-D Lookup Table17/1, 2-D Lookup Table16/1
  Switch7/1 -> Product13/2, Scope34/1
  Radians to Degrees12/1 -> Abs1/1
  Switch8/1 -> Product14/3
  Radians to Degrees13/1 -> Abs2/1
  Radians to Degrees17/1 -> Abs4/1
  Product13/1 -> Scope38/1, Sum18/1
  In2/1 -> Switch17/2, Radians to Degrees17/1, Radians to Degrees15/1, Switch7/2
  1-D Lookup Table73/1 -> Switch9/3
  2-D Lookup Table19/1 -> Switch8/1
  1-D Lookup Table72/1 -> Switch9/1
  Abs4/1 -> 1-D Lookup Table61/1
  Radians in1/1 -> Radians to Degrees13/1, Switch8/2, Radians to Degrees12/1, Switch9/2
  2-D Lookup Table18/1 -> Switch8/3
  Abs1/1 -> 1-D Lookup Table72/1
  2-D Lookup Table17/1 -> Switch17/1

== system simulink_flightgear_control_trim_wind_5/Plane/气动系数/Subsystem58/Subsystem28 ==
  Radians in : Inport
  Radians in1 : Inport  Port=2
  2-D Lookup Table23 : Lookup_n-D  BreakpointsForDimension1=dr  BreakpointsForDimension2=beta  Table=P3DAERO.delta_CM_25  InternalRulePriority=Speed  RndMeth=Simplest
      settings: InputPortMap=u0,u1
  2-D Lookup Table26 : Lookup_n-D  BreakpointsForDimension1=dr  BreakpointsForDimension2=beta  Table=P3DAERO.delta_CM_fu25  InternalRulePriority=Speed  RndMeth=Simplest
      settings: InputPortMap=u0,u1
  Abs1 : Abs  SaturateOnIntegerOverflow=off
  Gain25 : Gain  Gain=0.75
  Gain26 : Gain  Gain=0.75
  Radians to Degrees{23..25,32} (4 alike) : simulink_extras/Transformations/Radians to Degrees
  Saturation1 : Saturate  UpperLimit=15  LowerLimit=-15
  Saturation9 : Saturate  UpperLimit=15  LowerLimit=-15
  Scope16 : Scope
  Switch10 : Switch  SaturateOnIntegerOverflow=off  InputSameDT=off
  Out1 : Outport
  wires:
  2-D Lookup Table23/1 -> Gain25/1, Scope16/1
  Radians in/1 -> Radians to Degrees32/1, Switch10/2, Radians to Degrees24/1
  Radians in1/1 -> Radians to Degrees25/1, Radians to Degrees23/1
  Radians to Degrees23/1 -> Saturation9/1
  2-D Lookup Table26/1 -> Gain26/1
  Radians to Degrees25/1 -> Saturation1/1
  Radians to Degrees32/1 -> Abs1/1
  Gain26/1 -> Switch10/3
  Saturation9/1 -> 2-D Lookup Table23/2
  Gain25/1 -> Switch10/1
  Radians to Degrees24/1 -> 2-D Lookup Table23/1
  Switch10/1 -> Out1/1
  Abs1/1 -> 2-D Lookup Table26/1
  Saturation1/1 -> 2-D Lookup Table26/2

== system simulink_flightgear_control_trim_wind_5/Plane/气动系数/Subsystem58/Subsystem29 ==
  Radians in : Inport
  Radians in1 : Inport  Port=2
  2-D Lookup Table24 : Lookup_n-D  BreakpointsForDimension1=dr  BreakpointsForDimension2=beta  Table=P3DAERO.delta_CM_25  InternalRulePriority=Speed  RndMeth=Simplest
      settings: InputPortMap=u0,u1
  2-D Lookup Table25 : Lookup_n-D  BreakpointsForDimension1=dr  BreakpointsForDimension2=beta  Table=P3DAERO.delta_CM_fu25  InternalRulePriority=Speed  RndMeth=Simplest
      settings: InputPortMap=u0,u1
  Abs1 : Abs  SaturateOnIntegerOverflow=off
  Gain23 : Gain  Gain=0.25
  Gain24 : Gain  Gain=0.25
  Radians to Degrees{19..22} (4 alike) : simulink_extras/Transformations/Radians to Degrees
  Saturation10 : Saturate  UpperLimit=15  LowerLimit=-15
  Saturation2 : Saturate  UpperLimit=15  LowerLimit=-15
  Scope10 : Scope
  Switch13 : Switch  SaturateOnIntegerOverflow=off  InputSameDT=off
  Out1 : Outport
  wires:
  Radians to Degrees21/1 -> Saturation10/1
  2-D Lookup Table25/1 -> Gain24/1
  2-D Lookup Table24/1 -> Gain23/1
  Radians in1/1 -> Radians to Degrees19/1, Radians to Degrees21/1
  Saturation10/1 -> 2-D Lookup Table24/2
  Gain24/1 -> Switch13/3
  Radians to Degrees22/1 -> 2-D Lookup Table24/1
  Gain23/1 -> Scope10/1, Switch13/1
  Radians to Degrees20/1 -> Abs1/1
  Radians in/1 -> Radians to Degrees20/1, Switch13/2, Radians to Degrees22/1
  Abs1/1 -> 2-D Lookup Table25/1
  Saturation2/1 -> 2-D Lookup Table25/2
  Radians to Degrees19/1 -> Saturation2/1
  Switch13/1 -> Out1/1

== system simulink_flightgear_control_trim_wind_5/Plane/气动系数/Subsystem58/Subsystem3 ==
  note: k_alpha舵效
  note: 襟翼角度
  In1 : Inport
  Radians in : Inport  Port=2
  2-D Lookup Table8 : Lookup_n-D  BreakpointsForDimension1=flap  BreakpointsForDimension2=alpha  Table=P3DAERO.k_alpha  InternalRulePriority=Speed  RndMeth=Simplest
      settings: InputPortMap=u0,u1
  Radians to Degrees7 : simulink_extras/Transformations/Radians to Degrees
  Scope12 : Scope
  Out1 : Outport
  wires:
  In1/1 -> 2-D Lookup Table8/1
  2-D Lookup Table8/1 -> Out1/1, Scope12/1
  Radians to Degrees7/1 -> 2-D Lookup Table8/2
  Radians in/1 -> Radians to Degrees7/1

== system simulink_flightgear_control_trim_wind_5/Plane/气动系数/Subsystem58/Subsystem30 ==
  note: 高速模式
  note: 低速模式
  Radians in : Inport
  In2 : Inport  Port=2
  In3 : Inport  Port=3
  In4 : Inport  Port=4
  In5 : Inport  Port=5
  2-D Lookup Table3 : Lookup_n-D  BreakpointsForDimension1=high1  BreakpointsForDimension2=mach  Table=P3DAERO.delta_dot_CM_25_dot_alpha_highspeed  InternalRulePriority=Speed  RndMeth=Simplest
      settings: InputPortMap=u0,u1
  2-D Lookup Table4 : Lookup_n-D  BreakpointsForDimension1=flap  BreakpointsForDimension2=V_E  Table=P3DAERO.delta_dot_CM_25_dot_alpha_lowspeed  InternalRulePriority=Speed  RndMeth=Simplest
      settings: InputPortMap=u0,u1
  Gain10 : Gain  Gain=m2ft
  Product10 : Product
  Radians to Degrees6 : simulink_extras/Transformations/Radians to Degrees
  Scope25 : Scope
  Out1 : Outport
  wires:
  In2/1 -> 2-D Lookup Table4/1
  Gain10/1 -> 2-D Lookup Table3/1
  Product10/1 -> Out1/1
  2-D Lookup Table3/1 -> Product10/2, Scope25/1
  In4/1 -> Gain10/1
  Radians to Degrees6/1 -> Product10/1
  In5/1 -> 2-D Lookup Table3/2
  In3/1 -> 2-D Lookup Table4/2
  Radians in/1 -> Radians to Degrees6/1

== system simulink_flightgear_control_trim_wind_5/Plane/气动系数/Subsystem58/Subsystem31 ==
  In1 : Inport
  In2 : Inport  Port=2
  Constant5 : Constant  Value=0.25
  Gain : Gain  Gain=1/100
  Product : Product
  Scope3 : Scope
  Sum : Sum  Inputs=+-
  Out1 : Outport
  wires:
  Gain/1 -> Sum/1
  In1/1 -> Product/1
  Constant5/1 -> Sum/2
  Sum/1 -> Product/2
  In2/1 -> Gain/1
  Product/1 -> Out1/1, Scope3/1

== system simulink_flightgear_control_trim_wind_5/Plane/气动系数/Subsystem58/Subsystem32 ==
  note: 迎角角速度rad/s
  note: 平均气动弦长ft
  note: 速度ft/s
  u : Inport
  In2 : Inport  Port=2
  In3 : Inport  Port=3
  In4 : Inport  Port=4
  In5 : Inport  Port=5
  2-D Lookup Table5 : Lookup_n-D  BreakpointsForDimension1=high2  BreakpointsForDimension2=mach  Table=P3DAERO.dot_CM_25_dot_alpha_dian  InternalRulePriority=Speed  RndMeth=Simplest
      settings: InputPortMap=u0,u1
  Constant8 : Constant  Value=2
  Constant9 : Constant  Value=27.3
  Divide : Product  Inputs=**//
  Gain : Gain
  Gain4 : Gain  Gain=m2ft
  MATLAB Function15 : MATLAB Function  TreatAsAtomicUnit=on
  Product2 : Product  Inputs=3
  Scope4 : Scope
  Scope9 : Scope
  Out1 : Outport
  wires:
  Gain4/1 -> 2-D Lookup Table5/1
  Constant8/1 -> Divide/4
  Product2/1 -> Gain/1
  In4/1 -> Divide/1
  Constant9/1 -> Divide/2
  Divide/1 -> Scope4/1, Product2/3
  2-D Lookup Table5/1 -> Product2/2
  MATLAB Function15/1(y) -> Product2/1
  In3/1 -> 2-D Lookup Table5/2
  In2/1 -> Gain4/1
  u/1 -> MATLAB Function15/1(u)
  In5/1 -> Divide/3
  Gain/1 -> Out1/1, Scope9/1

== system simulink_flightgear_control_trim_wind_5/Plane/气动系数/Subsystem58/Subsystem33 ==
  note: 速度ft/s
  note: 平均气动弦长ft
  note: q滚转角速度rad/s
  In1 : Inport
  In2 : Inport  Port=2
  In3 : Inport  Port=3
  In4 : Inport  Port=4
  2-D Lookup Table6 : Lookup_n-D  BreakpointsForDimension1=high2  BreakpointsForDimension2=mach  Table=P3DAERO.dot_CM_25_dot_q  InternalRulePriority=Speed  RndMeth=Simplest
      settings: InputPortMap=u0,u1
  Constant12 : Constant  Value=2
  Constant15 : Constant  Value=27.3
  Divide1 : Product  Inputs=**//
  Gain5 : Gain  Gain=m2ft
  Product3 : Product
  Scope5 : Scope
  Scope7 : Scope
  Out1 : Outport
  wires:
  Product3/1 -> Out1/1, Scope7/1
  Constant15/1 -> Divide1/2
  Gain5/1 -> 2-D Lookup Table6/1
  In2/1 -> 2-D Lookup Table6/2
  2-D Lookup Table6/1 -> Scope5/1, Product3/1
  Divide1/1 -> Product3/2
  Constant12/1 -> Divide1/4
  In1/1 -> Gain5/1
  In3/1 -> Divide1/1
  In4/1 -> Divide1/3

== system simulink_flightgear_control_trim_wind_5/Plane/气动系数/Subsystem58/Subsystem34 ==
  note: 法向过载
  note: 低速模式
  note: 高速模式
  In1 : Inport
  In2 : Inport  Port=2
  In3 : Inport  Port=3
  In4 : Inport  Port=4
  In5 : Inport  Port=5
  2-D Lookup Table7 : Lookup_n-D  BreakpointsForDimension1=high1  BreakpointsForDimension2=mach  Table=P3DAERO.dot_CM_25_dot_nz_highspeed  InternalRulePriority=Speed  RndMeth=Simplest
      settings: InputPortMap=u0,u1
  2-D Lookup Table9 : Lookup_n-D  BreakpointsForDimension1=flap  BreakpointsForDimension2=V_E  Table=P3DAERO.dot_CM_25_dot_nz_lowspeed  InternalRulePriority=Speed  RndMeth=Simplest
      settings: InputPortMap=u0,u1
  Gain8 : Gain  Gain=m2ft
  Product1 : Product
  Scope29 : Scope
  Out1 : Outport
  wires:
  2-D Lookup Table7/1 -> Product1/2, Scope29/1
  Product1/1 -> Out1/1
  In2/1 -> 2-D Lookup Table9/1
  Gain8/1 -> 2-D Lookup Table7/1
  In5/1 -> 2-D Lookup Table7/2
  In1/1 -> Product1/1
  In4/1 -> Gain8/1
  In3/1 -> 2-D Lookup Table9/2

== system simulink_flightgear_control_trim_wind_5/Plane/气动系数/Subsystem58/Subsystem35 ==
  note: dot_CM_dot_delta
  note: 高速模式
  In1 : Inport
  In2 : Inport  Port=2
  In3 : Inport  Port=3
  Radians in : Inport  Port=4
  2-D Lookup Table10 : Lookup_n-D  BreakpointsForDimension1=high1  BreakpointsForDimension2=mach  Table=P3DAERO.dot_CM_dot_delta  InternalRulePriority=Speed  RndMeth=Simplest
      settings: InputPortMap=u0,u1
  Gain20 : Gain  Gain=m2ft
  Product5 : Product  Inputs=3
  Radians to Degrees3 : simulink_extras/Transformations/Radians to Degrees
  Scope17 : Scope
  Out1 : Outport
  wires:
  In2/1 -> Gain20/1
  In3/1 -> 2-D Lookup Table10/2
  In1/1 -> Product5/1
  2-D Lookup Table10/1 -> Product5/2
  Gain20/1 -> 2-D Lookup Table10/1
  Radians to Degrees3/1 -> Product5/3
  Product5/1 -> Out1/1, Scope17/1
  Radians in/1 -> Radians to Degrees3/1

== system simulink_flightgear_control_trim_wind_5/Plane/气动系数/Subsystem58/Subsystem36 ==
  note: dot_CM_dot_delta_ei
  In1 : Inport
  In2 : Inport  Port=2
  In3 : Inport  Port=3
  Radians in : Inport  Port=4
  2-D Lookup Table11 : Lookup_n-D  BreakpointsForDimension1=high1  BreakpointsForDimension2=mach  Table=P3DAERO.dot_CM_delta_ei  InternalRulePriority=Speed  RndMeth=Simplest
      settings: InputPortMap=u0,u1
  Gain21 : Gain  Gain=m2ft
  Product6 : Product  Inputs=3
  Radians to Degrees1 : simulink_extras/Transformations/Radians to Degrees
  Scope18 : Scope
  Out1 : Outport
  wires:
  Product6/1 -> Out1/1, Scope18/1
  In1/1 -> Product6/1
  In3/1 -> 2-D Lookup Table11/2
  In2/1 -> Gain21/1
  Gain21/1 -> 2-D Lookup Table11/1
  2-D Lookup Table11/1 -> Product6/2
  Radians to Degrees1/1 -> Product6/3
  Radians in/1 -> Radians to Degrees1/1

== system simulink_flightgear_control_trim_wind_5/Plane/气动系数/Subsystem58/Subsystem37 ==
  note: dot_CM_dot_delta_eo
  In1 : Inport
  In2 : Inport  Port=2
  In3 : Inport  Port=3
  Radians in : Inport  Port=4
  2-D Lookup Table12 : Lookup_n-D  BreakpointsForDimension1=high1  BreakpointsForDimension2=mach  Table=P3DAERO.dot_CM_delta_eo  InternalRulePriority=Speed  RndMeth=Simplest
      settings: InputPortMap=u0,u1
  Gain22 : Gain  Gain=m2ft
  Product7 : Product  Inputs=3
  Radians to Degrees5 : simulink_extras/Transformations/Radians to Degrees
  Scope19 : Scope
  Out1 : Outport
  wires:
  Radians to Degrees5/1 -> Product7/3
  2-D Lookup Table12/1 -> Product7/2
  Product7/1 -> Out1/1, Scope19/1
  Gain22/1 -> 2-D Lookup Table12/1
  Radians in/1 -> Radians to Degrees5/1
  In3/1 -> 2-D Lookup Table12/2
  In2/1 -> Gain22/1
  In1/1 -> Product7/1

== system simulink_flightgear_control_trim_wind_5/Plane/气动系数/Subsystem58/Subsystem38 ==
  In1 : Inport
  In2 : Inport  Port=2
  Radians in : Inport  Port=3
  In4 : Inport  Port=4
  1-D Lookup Table91 : Lookup_n-D  NumberOfTableDimensions=1  BreakpointsForDimension1=P3DAERO.delta_CM_25_landinggear_mach(1,:)  Table=P3DAERO.delta_CM_25_landinggear_mach(2,:)  InternalRulePriority=Speed  RndMeth=Simplest
  2-D Lookup Table20 : Lookup_n-D  BreakpointsForDimension1=flap  BreakpointsForDimension2=alpha  Table=P3DAERO.delta_CM_25_landinggear  InternalRulePriority=Speed  RndMeth=Simplest
      settings: InputPortMap=u0,u1
  Product15 : Product  Inputs=3
  Radians to Degrees11 : simulink_extras/Transformations/Radians to Degrees
  Scope47 : Scope
  Out1 : Outport
  wires:
  2-D Lookup Table20/1 -> Product15/2
  Radians in/1 -> Radians to Degrees11/1
  Radians to Degrees11/1 -> 2-D Lookup Table20/2
  In2/1 -> 2-D Lookup Table20/1
  In1/1 -> Product15/1
  In4/1 -> 1-D Lookup Table91/1
  Product15/1 -> Out1/1, Scope47/1
  1-D Lookup Table91/1 -> Product15/3

== system simulink_flightgear_control_trim_wind_5/Plane/气动系数/Subsystem58/Subsystem39 ==
  note: 米变英尺
  note: n beta地效修正
  In1 : Inport
  In2 : Inport  Port=2
  Radians in : Inport  Port=3
  In4 : Inport  Port=4
  1-D Lookup Table97 : Lookup_n-D  NumberOfTableDimensions=1  BreakpointsForDimension1=P3DAERO.k_ge(1,:)  Table=P3DAERO.k_ge(2,:)  InternalRulePriority=Speed  RndMeth=Simplest
  2-D Lookup Table : Lookup_n-D  BreakpointsForDimension1=flap  BreakpointsForDimension2=alpha  Table=P3DAERO.dot_CN_dot_beta  InternalRulePriority=Speed  RndMeth=Simplest
      settings: InputPortMap=u0,u1
  2-D Lookup Table1 : Lookup_n-D  BreakpointsForDimension1=high1  BreakpointsForDimension2=mach  Table=P3DAERO.dot_CN_dot_beta_mach  InternalRulePriority=Speed  RndMeth=Simplest
      settings: InputPortMap=u0,u1
  2-D Lookup Table2 : Lookup_n-D  BreakpointsForDimension1=flap  BreakpointsForDimension2=alpha1  Table=P3DAERO.Fn_beta  InternalRulePriority=Speed  RndMeth=Simplest
      settings: InputPortMap=u0,u1
  Constant21 : Constant
  Gain14 : Gain  Gain=m2ft
  Gain4 : Gain  Gain=m2ft
  Product16 : Product
  Product9 : Product  Inputs=3
  Radians to Degrees24 : simulink_extras/Transformations/Radians to Degrees
  Radians to Degrees4 : simulink_extras/Transformations/Radians to Degrees
  Saturation5 : Saturate  UpperLimit=14  LowerLimit=0
  Scope31 : Scope
  Sum11 : Sum
  Switch5 : Switch  Criteria=u2 > Threshold  Threshold=24  SaturateOnIntegerOverflow=off  InputSameDT=off
  Out1 : Outport
  wires:
  2-D Lookup Table1/1 -> Product9/3
  Radians to Degrees4/1 -> Saturation5/1
  2-D Lookup Table/1 -> Product9/2
  2-D Lookup Table2/1 -> Product16/2
  Switch5/1 -> Product9/1, Scope31/1
  In1/1 -> Switch5/2, Gain14/1, Gain4/1
  Saturation5/1 -> 2-D Lookup Table2/2
  1-D Lookup Table97/1 -> Product16/1
  Radians in/1 -> Radians to Degrees4/1, Radians to Degrees24/1
  Gain4/1 -> 2-D Lookup Table1/1
  Radians to Degrees24/1 -> 2-D Lookup Table/2
  Constant21/1 -> Sum11/1, Switch5/1
  Product16/1 -> Sum11/2
  Sum11/1 -> Switch5/3
  Gain14/1 -> 1-D Lookup Table97/1
  In2/1 -> 2-D Lookup Table2/1, 2-D Lookup Table/1
  In4/1 -> 2-D Lookup Table1/2
  Product9/1 -> Out1/1

== system simulink_flightgear_control_trim_wind_5/Plane/气动系数/Subsystem58/Subsystem4 ==
  note: 高速模式
  note: 低速模式
  Radians in : Inport
  In2 : Inport  Port=2
  In3 : Inport  Port=3
  In4 : Inport  Port=4
  In5 : Inport  Port=5
  2-D Lookup Table2 : Lookup_n-D  BreakpointsForDimension1=flap  BreakpointsForDimension2=V_E  Table=P3DAERO.delta_dot_CL_dot_alpha_lowspeed  InternalRulePriority=Speed  RndMeth=Simplest
      settings: InputPortMap=u0,u1
  2-D Lookup Table21 : Lookup_n-D  BreakpointsForDimension1=high1  BreakpointsForDimension2=mach  Table=P3DAERO.delta_dot_CL_dot_alpha_highspeed  InternalRulePriority=Speed  RndMeth=Simplest
      settings: InputPortMap=u0,u1
  Product1 : Product
  Radians to Degrees1 : simulink_extras/Transformations/Radians to Degrees
  Scope3 : Scope  NumInputPorts=2
  Velocity Conversion : aerolibconvert2/Velocity Conversion  IU=m/s  OU=ft/s
  Out1 : Outport
  wires:
  Radians in/1 -> Radians to Degrees1/1
  In2/1 -> 2-D Lookup Table2/1
  In4/1 -> Velocity Conversion/1
  2-D Lookup Table21/1 -> Scope3/2, Product1/2
  Radians to Degrees1/1 -> Product1/1
  In3/1 -> 2-D Lookup Table2/2
  Product1/1 -> Out1/1, Scope3/1
  In5/1 -> 2-D Lookup Table21/2
  Velocity Conversion/1 -> 2-D Lookup Table21/1

== system simulink_flightgear_control_trim_wind_5/Plane/气动系数/Subsystem58/Subsystem40 ==
  note: 平均气动弦长ft
  note: 展长ft
  In1 : Inport
  Radians in : Inport  Port=2
  In3 : Inport  Port=3
  2-D Lookup Table3 : Lookup_n-D  BreakpointsForDimension1=flap  BreakpointsForDimension2=alpha  Table=P3DAERO.dot_CC_dot_beta  InternalRulePriority=Speed  RndMeth=Simplest
      settings: InputPortMap=u0,u1
  Constant10 : Constant  Value=0.25
  Constant12 : Constant  Value=195.7
  Constant5 : Constant  Value=27.3
  Divide1 : Product  Inputs=*/
  Gain : Gain  Gain=1/100
  Product3 : Product  Inputs=3
  Radians to Degrees6 : simulink_extras/Transformations/Radians to Degrees
  Sum : Sum  Inputs=+-
  Out1 : Outport
  wires:
  Sum/1 -> Product3/2
  Constant12/1 -> Divide1/2
  Gain/1 -> Sum/1
  Radians to Degrees6/1 -> 2-D Lookup Table3/2
  2-D Lookup Table3/1 -> Product3/1
  Product3/1 -> Out1/1
  Divide1/1 -> Product3/3
  In1/1 -> 2-D Lookup Table3/1
  Constant5/1 -> Divide1/1
  Constant10/1 -> Sum/2
  In3/1 -> Gain/1
  Radians in/1 -> Radians to Degrees6/1
